simulink model "quadruped_wbc"  (R2026b)
settings: Solver=ode23t  StopTime=22.4  MaxStep=0.005  RelTol=2e-3  AbsTol=2e-4
values from neighbouring files (symbols this model uses):
  s = min(max(s, 0.0), 1.0)    [gait_swing_controller.m]
undefined symbols (not defined in the file or in its folder): X, Y, Z
libraries: sm_lib x84, nesl_utility x46
(part 2 of 2)

== matlab function quadruped_wbc/WBC_Controller ==
  data: t input; tau_legs output; p_com input; v_com input; quat_wb input; omega_w input; q_legs input; dq_legs input; gait_mode input; p_box input; v_box input; tau_arm output; rpy output; F_grf output; contact_mask output; nav_log output; wrench_assist output; F_suction output; q_arm output; w_arm output; mission_log output
function [tau_legs, tau_arm, rpy, F_grf, contact_mask, nav_log, wrench_assist, F_suction, q_arm, w_arm, mission_log] = ...
    wbc_control_fcn(t, p_com, v_com, quat_wb, omega_w, q_legs, dq_legs, gait_mode, p_box, v_box)
%WBC_CONTROL_FCN Closed-loop VMC + Raibert + Pure-Pursuit + 6-Axis Arm Pick-and-Place.
coder.extrinsic('wbc_step');
tau_legs      = zeros(8, 1);
tau_arm       = zeros(6, 1);
rpy           = zeros(3, 1);
F_grf         = zeros(12, 1);
contact_mask  = ones(4, 1);
nav_log       = zeros(12, 1);
wrench_assist = zeros(6, 1);
F_suction     = zeros(3, 1);
q_arm         = zeros(6, 1);
w_arm         = zeros(6, 1);
mission_log   = zeros(8, 1);
[tau_legs, tau_arm, rpy, F_grf, contact_mask, nav_log, wrench_assist, F_suction, q_arm, w_arm, mission_log] = ...
    wbc_step(t, p_com, v_com, quat_wb, omega_w, q_legs, dq_legs, gait_mode, p_box, v_box);
end
